simulink model "afe_inv_psm_with_hf_models"  (R2026a)
settings: Solver=ode23tb  StopTime=simlength  FixedStep=tc  MaxStep=glb_time.tc
values from neighbouring files (symbols this model uses):
  afe_ctrl = ctrl_afe_setup(glb_time.ts_afe, grid_emu.omega_grid_nom)    [init_model.m]
  afe_pwm_phase_shift_mod1 = 0    [init_model.m]
  CTRPIFF_CLIP_RELEASE = 0.001    [init_model.m]
  DThs_init = 0    [init_model.m]
  filters = setup_global_filters(glb_time.ts_afe, glb_time.ts_inv, glb_time.ts_dab, glb_time.tc)    [init_model.m]
  frt_data = frt_settings(test_index, test_subindex, asymmetric_error_type,      enable_frt_1, enable_frt_2, start_time_LVRT, deepPOSxi, deepPOSeta, deepNEGxi, deepNEGeta)    [init_model.m]
  glb_time = timing_setup(fpwm_afe, trgo_afe, fpwm_inv, trgo_inv, fpwm_single_phase_inv, trgo_single_phase_inv, fpwm_dab, trgo_dab,      fpwm_psfbc, trgo_psfbc, fpwm_isop_rail, trgo_isop_rail, fpwm_cllc, trgo_cllc, t_measure, tc_factor, tc_decimation, delay_pwm, dead_time_afe,      dead_time_inv, dead_time_single_phase_inv, dead_time_dab, dead_time_psfbc, dead_time_isop_rail, dead_time_cllc)    [init_model.m]
  grid_emu = grid_three_phase_emulator('Dyn11', delta_star, grid_nominal_power, application_voltage, us1, us2, fgrid,                  eq_grid_inductance, eq_grid_resistance, eta, ucc, i1m, p_iron, n1, n2, core_area, core_length, mur,                  up_xi_pu_ref, up_eta_pu_ref, un_xi_pu_ref, un_eta_pu_ref)    [init_model.m]
  i_react_pos_ref_2 = -ixi_ref_mod1*tan(acos(0.95))    [init_model.m]
  i_react_pos_ref_3 = ixi_ref_mod1*tan(acos(0.95))    [init_model.m]
  inv_pwm_phase_shift_mod1 = 0    [init_model.m]
  ixi_ref_mod1 = -0.85    [init_model.m]
  ki_align = 18    [init_model.m]
  kp_align = 0.25    [init_model.m]
  lim_down_align = -0.05    [init_model.m]
  lim_up_align = 0.05    [init_model.m]
  mavarage_filter_frequency_base_order = 2    [init_model.m]
  omega_m_sim = psm.omega_m_bez    [init_model.m]
  psm = psm_calculus_with_variants(application_voltage)    [init_model.m]
  psm_ctrl = ctrl_pmsm_setup(glb_time.ts_inv, psm.omega_bez, u_psm_scale, psm.Jm_norm)    [init_model.m]
  rms_tc = rms_filter_setup(rms_tc_obj)    [init_model.m]
  simlength = 1.75    [init_model.m]
  Tambient = 40    [init_model.m]
  time_aux_power_supply_fault = 1e3    (= 1000)    [init_model.m]
  time_gain_afe_module_1 = 1.0002    [init_model.m]
  time_gain_inv_module_2 = 1.001    [init_model.m]
  time_i_react_pos_ref_1 = start_time_LVRT + error_length + 0.335    [init_model.m]
  time_i_react_pos_ref_2 = time_i_react_pos_ref_1 + 0.5    (= 0.5)    [init_model.m]
  time_start_motor_control = 0.25    [init_model.m]
  torque_overload_factor = 1    [init_model.m]
  u_cm_comp_mod1 = 0    [init_model.m]
  u_psm_scale_ekf = sqrt(3)/2 * 2/3 * hwdata.inv.udc_nom/psm.ubez    [init_model.m]
undefined symbols (not defined in the file or in its folder): hf_power_cable_model, hwdata, magnitude, omega_m_bez, rpm_base, torque_base
libraries: fl_lib x136, nesl_utility x57, moving_average_filter x10, moving_average_filter_cc x8, ee_lib x5, sl_discontinuities x3, single_phase_transformer_lib x3, linear_double_integrator_observer_ccaller x2, discrete_time_low_pass_filter x2, threephase_inductor_lib x2, three_phase_pwm_modulator x2, three_phase_inverter_ideal_switch_based_model x2
(part 2 of 10)

== system afe_inv_psm_with_hf_models/grid/grid_emulator ==
  3ph_Dyg : Subsystem
  Bus Selector : BusSelector  OutputSignals=ua_grid_emu,ub_grid_emu,uc_grid_emu
  Bus Selector1 : BusSelector  OutputSignals=gamma_grid_emulator,omega_grid_emulator
  Controlled Voltage Source : fl_lib/Electrical/Electrical Sources/Controlled Voltage Source
  Controlled Voltage Source1 : fl_lib/Electrical/Electrical Sources/Controlled Voltage Source
  Controlled Voltage Source2 : fl_lib/Electrical/Electrical Sources/Controlled Voltage Source
  Electrical Reference : fl_lib/Electrical/Electrical Elements/Electrical Reference
  Simulink-PS Converter : nesl_utility/Simulink-PS Converter  PhysicalDomain=network_engine_domain  SubClassName=ps_input  LeftPortType=input  RightPortType=output  PseudoPeriodic=off  Frequencies=[]  NoiseDistribution=none  NoiseParameters=[]  Unit=V  AffineConversion=on  FilteringAndDerivatives=provide  SimscapeFilterOrder=1  InputFilterTimeConstant=0.001  UdotUserProvided=0
  Simulink-PS Converter1 : nesl_utility/Simulink-PS Converter  PhysicalDomain=network_engine_domain  SubClassName=ps_input  LeftPortType=input  RightPortType=output  PseudoPeriodic=off  Frequencies=[]  NoiseDistribution=none  NoiseParameters=[]  Unit=V  AffineConversion=on  FilteringAndDerivatives=provide  SimscapeFilterOrder=1  InputFilterTimeConstant=0.001  UdotUserProvided=0
  Simulink-PS Converter2 : nesl_utility/Simulink-PS Converter  PhysicalDomain=network_engine_domain  SubClassName=ps_input  LeftPortType=input  RightPortType=output  PseudoPeriodic=off  Frequencies=[]  NoiseDistribution=none  NoiseParameters=[]  Unit=V  AffineConversion=on  FilteringAndDerivatives=provide  SimscapeFilterOrder=1  InputFilterTimeConstant=0.001  UdotUserProvided=0
  Solver Configuration : nesl_utility/Solver Configuration  PhysicalDomain=network_engine_domain  SubClassName=solver  LeftPortType=input  RightPortType=generic  Tones=[]  Harmonics=[]  SimulateNoise=off  Profile=off  UseLocalSampling=off  EnableSwitchedLinearOptims=on  FrequencyDomain=off  UseCCode=off  RelTol=0.001  AbsTol=0.001  MinStep=1e-09  ToWorkspace=off  RevertToSquareIcSolve=off  NumHomotopyIterations=100  PhasorMode=off  PhasorModeNumHarmonics=1  ConsistencySolver=NEWTON_FTOL  CanonicalOrdering=UNORDERED  OptimizeIntermediates=UNOPTIMIZED  IndexReductionMethod=DerivativeReplacement  DoDC=on  ResidualTolerance=1e-09  ConsistencyTolSource=GLOBAL  ConsistencyAbsTol=0.001  ConsistencyRelTol=0.001  ConsistencyTolFactor=0.001  UseLocalSolver=on  LocalSolverChoice=NE_BACKWARD_EULER_ADVANCER  ResolveIndetEquations=on  FunctionEvalNumThread=1  LocalSolverSampleTime=glb_time.tc  DoFixedCost=on  MaxNonlinIter=nonlinear_iterations  MaxModeIter=2  ComputeImpulses=off  ImpulseIterations=2  LinearAlgebra=auto  LinearAlgebraNumThread=0  EquationFormulation=NE_TIME_EF  DelaysMemoryBudget=1024  AutomaticFiltering=on  FilteringTimeConstant=0.001  PartitionStorageMethod=AS_NEEDED  PartitionMemoryBudget=1024  PartitionMethod=ROBUST  MultibodyUseLocalSolver=off  MultibodyLocalSolverChoice=ODE1  MultibodyLocalSolverSampleTime=0.001
  three_phase_voltage_source_with_frt_emulator : three_phase_voltage_with_frt_emulator/three_phase_voltage_source_with_frt_emulator  nominal_frequency_m=grid_emu.fgrid_nom  nominal_voltage_m=grid_emu.us_primary_nom  Vemu_ref_norm_m=grid_emu.Vemu_ref_norm  vp_xi_pu_m=grid_emu.up_xi_pu_ref  vp_eta_pu_m=grid_emu.up_eta_pu_ref  vn_xi_pu_m=grid_emu.un_xi_pu_ref  vn_eta_pu_m=grid_emu.un_eta_pu_ref  Am=filters.afe.SOF_50Hz.ss_c.A  Bm=filters.afe.SOF_50Hz.ss_c.B  Cm=filters.afe.SOF_50Hz.ss_c.C  enable_frt_1_m=frt_data.enable_frt_1  enable_frt_2_m=frt_data.enable_frt_2  start_time_LVRT_m=frt_data.start_time_LVRT  end_time_LVRT_m=frt_data.end_time_LVRT  deepPOSxi_m=frt_data.deepPOSxi  deepPOSeta_m=frt_data.deepPOSeta  deepNEGxi_m=frt_data.deepNEGxi  deepNEGeta_m=frt_data.deepNEGeta  Amplitude_U_m=frt_data.Amplitude_U  Amplitude_V_m=frt_data.Amplitude_V  Amplitude_W_m=frt_data.Amplitude_W  t_ramp_m=frt_data.t_ramp  Phase_shift_m=frt_data.Phase_shift
  threephase_vi_measures : Subsystem
  u1 : PMIOPort  Side=Right
  u2 : PMIOPort  Port=2  Side=Right
  u3 : PMIOPort  Port=3  Side=Right
  tag scope: gamma_grid_emulator=global, omega_grid_emulator=global
  wires:
  Bus Selector1/2 -> [omega_grid_emulator]  "<omega_grid_emulator>"
  Bus Selector1/1 -> [gamma_grid_emulator]  "<gamma_grid_emulator>"
  Bus Selector/2 -> Simulink-PS Converter1/1  "<ub_grid_emu>"
  Bus Selector/3 -> Simulink-PS Converter2/1  "<uc_grid_emu>"
  three_phase_voltage_source_with_frt_emulator/1 -> Bus Selector1/1, Bus Selector/1
  Bus Selector/1 -> Simulink-PS Converter/1  "<ua_grid_emu>"
  connections:
  Simulink-PS Converter/RConn1 -- Controlled Voltage Source/RConn1
  Simulink-PS Converter1/RConn1 -- Controlled Voltage Source1/RConn1
  Simulink-PS Converter2/RConn1 -- Controlled Voltage Source2/RConn1
  Electrical Reference/LConn1 -- Controlled Voltage Source/RConn2 -- Controlled Voltage Source1/RConn2 -- Controlled Voltage Source2/RConn2 -- Solver Configuration/RConn1
  3ph_Dyg/RConn1 -- u1/RConn1
  3ph_Dyg/RConn2 -- u2/RConn1
  3ph_Dyg/RConn3 -- u3/RConn1
  3ph_Dyg/LConn1 -- threephase_vi_measures/RConn1
  3ph_Dyg/LConn2 -- threephase_vi_measures/RConn2
  3ph_Dyg/LConn3 -- threephase_vi_measures/RConn3
  Controlled Voltage Source/LConn1 -- threephase_vi_measures/LConn1
  Controlled Voltage Source1/LConn1 -- threephase_vi_measures/LConn2
  Controlled Voltage Source2/LConn1 -- threephase_vi_measures/LConn3

== system afe_inv_psm_with_hf_models/grid/threephase_vi_measures ==
  Bus Creator : BusCreator  Inputs=6
  Current Sensor : fl_lib/Electrical/Electrical Sensors/Current Sensor
  Current Sensor1 : fl_lib/Electrical/Electrical Sensors/Current Sensor
  Current Sensor2 : fl_lib/Electrical/Electrical Sensors/Current Sensor
  Electrical Reference1 : fl_lib/Electrical/Electrical Elements/Electrical Reference
  Selector : Selector  InputPortWidth=6  IndexOptions=Index vector (dialog)  Indices=[1 2 3]  OutputSizes=1
  Selector1 : Selector  InputPortWidth=6  IndexOptions=Index vector (dialog)  Indices=[4 5 6]  OutputSizes=1
  Voltage Sensor : fl_lib/Electrical/Electrical Sensors/Voltage Sensor
  Voltage Sensor1 : fl_lib/Electrical/Electrical Sensors/Voltage Sensor
  Voltage Sensor2 : fl_lib/Electrical/Electrical Sensors/Voltage Sensor
  ia_grid : nesl_utility/PS-Simulink Converter  PhysicalDomain=network_engine_domain  SubClassName=ps_output  LeftPortType=input  RightPortType=output  PseudoPeriodic=off  Frequencies=[]  VectorFormat=1-D array  Unit=A  AffineConversion=off
  ib_grid : nesl_utility/PS-Simulink Converter  PhysicalDomain=network_engine_domain  SubClassName=ps_output  LeftPortType=input  RightPortType=output  PseudoPeriodic=off  Frequencies=[]  VectorFormat=1-D array  Unit=A  AffineConversion=off
  ic_grid : nesl_utility/PS-Simulink Converter  PhysicalDomain=network_engine_domain  SubClassName=ps_output  LeftPortType=input  RightPortType=output  PseudoPeriodic=off  Frequencies=[]  VectorFormat=1-D array  Unit=A  AffineConversion=off
  ig_abc/ug_abc : Scope  NumInputPorts=2
      settings: SampleTime=glb_time.tc  ActiveDisplayYMinimum=-728.92703752654245  ActiveDisplayYMaximum=734.90808013997  DataLoggingVariableName=ScopeData2
  ua_grid : nesl_utility/PS-Simulink Converter  PhysicalDomain=network_engine_domain  SubClassName=ps_output  LeftPortType=input  RightPortType=output  PseudoPeriodic=off  Frequencies=[]  VectorFormat=1-D array  Unit=V  AffineConversion=off
  ub_grid : nesl_utility/PS-Simulink Converter  PhysicalDomain=network_engine_domain  SubClassName=ps_output  LeftPortType=input  RightPortType=output  PseudoPeriodic=off  Frequencies=[]  VectorFormat=1-D array  Unit=V  AffineConversion=off
  uc_grid : nesl_utility/PS-Simulink Converter  PhysicalDomain=network_engine_domain  SubClassName=ps_output  LeftPortType=input  RightPortType=output  PseudoPeriodic=off  Frequencies=[]  VectorFormat=1-D array  Unit=V  AffineConversion=off
  Ua : PMIOPort  Side=Left
  ua : PMIOPort  Port=2  Side=Right
  Ub : PMIOPort  Port=3  Side=Left
  ub : PMIOPort  Port=4  Side=Right
  Uc : PMIOPort  Port=5  Side=Left
  uc : PMIOPort  Port=6  Side=Right
  tag scope: ig_abc=global, ug_abc=global
  wires:
  Bus Creator/1 -> Selector1/1, Selector/1  "vi_data"
  Selector/1 -> [ug_abc]
  ib_grid/1 -> Bus Creator/5  "ib"
  ia_grid/1 -> Bus Creator/4  "ia"
  ic_grid/1 -> Bus Creator/6  "ic"
  ua_grid/1 -> Bus Creator/1  "ua"
  ub_grid/1 -> Bus Creator/2  "ub"
  uc_grid/1 -> Bus Creator/3  "uc"
  Selector1/1 -> [ig_abc]
  [ug_abc] -> ig_abc/ug_abc/2  "ug_abc(line)"
  [ig_abc] -> ig_abc/ug_abc/1  "ig_abc(line)"
  connections:
  Current Sensor1/LConn1 -- Ub/RConn1 -- Voltage Sensor1/LConn1
  Electrical Reference1/LConn1 -- Voltage Sensor/RConn2 -- Voltage Sensor2/RConn2 -- Voltage Sensor1/RConn2
  Voltage Sensor/RConn1 -- ua_grid/LConn1
  Current Sensor/RConn2 -- ua/RConn1
  Voltage Sensor1/RConn1 -- ub_grid/LConn1
  Voltage Sensor2/LConn1 -- Current Sensor2/LConn1 -- Uc/RConn1
  Current Sensor/LConn1 -- Ua/RConn1 -- Voltage Sensor/LConn1
  Current Sensor1/RConn2 -- ub/RConn1
  Voltage Sensor2/RConn1 -- uc_grid/LConn1
  ib_grid/LConn1 -- Current Sensor1/RConn1
  ia_grid/LConn1 -- Current Sensor/RConn1
  ic_grid/LConn1 -- Current Sensor2/RConn1
  Current Sensor2/RConn2 -- uc/RConn1

== system afe_inv_psm_with_hf_models/inverter_measurement_sim/high_frequency_power_cable ==
  To Workspace21 : ToWorkspace  VariableName=is_uvw_cm_sim  SampleTime=glb_time.tc
      settings: MaxDataPoints=glb_time.Nc
  To Workspace22 : ToWorkspace  VariableName=udc_pgnd_sim  SampleTime=glb_time.tc
      settings: MaxDataPoints=glb_time.Nc
  To Workspace23 : ToWorkspace  VariableName=udc_ngnd_sim  SampleTime=glb_time.tc
      settings: MaxDataPoints=glb_time.Nc
  To Workspace24 : ToWorkspace  VariableName=iz_power_cable_drive_side_sim  SampleTime=glb_time.tc
      settings: MaxDataPoints=glb_time.Nc
  To Workspace25 : ToWorkspace  VariableName=i_power_cable_drive_side_sim  SampleTime=glb_time.tc
      settings: MaxDataPoints=glb_time.Nc
  To Workspace26 : ToWorkspace  VariableName=u_power_cable_drive_side_sim  SampleTime=glb_time.tc
      settings: MaxDataPoints=glb_time.Nc
  To Workspace27 : ToWorkspace  VariableName=iz_power_cable_machine_side_sim  SampleTime=glb_time.tc
      settings: MaxDataPoints=glb_time.Nc
  To Workspace28 : ToWorkspace  VariableName=i_power_cable_machine_side_sim  SampleTime=glb_time.tc
      settings: MaxDataPoints=glb_time.Nc
  To Workspace29 : ToWorkspace  VariableName=u_power_cable_machine_side_sim  SampleTime=glb_time.tc
      settings: MaxDataPoints=glb_time.Nc
  wires:
  [i_power_cable_drive_side] -> To Workspace25/1  "i_power_cable_drive_side"
  [is_uvw_cm] -> To Workspace21/1  "is_uvw_cm"
  [iz_power_cable_machine_side] -> To Workspace27/1  "iz_power_cable_machine_side"
  [iz_power_cable_drive_side] -> To Workspace24/1  "iz_power_cable_drive_side"
  [i_power_cable_machine_side] -> To Workspace28/1  "i_power_cable_machine_side"
  [udc_pgnd] -> To Workspace22/1  "udc_pgnd"
  [u_power_cable_drive_side] -> To Workspace26/1  "u_power_cable_drive_side"
  [udc_ngnd] -> To Workspace23/1  "udc_ngnd"
  [u_power_cable_machine_side] -> To Workspace29/1  "u_power_cable_machine_side"

== system afe_inv_psm_with_hf_models/inverter_measurement_sim/module_1 ==
  To Workspace12 : ToWorkspace  VariableName=ileg_dc_inv_sim_mod1  SampleTime=glb_time.tc
      settings: MaxDataPoints=glb_time.Nc
  To Workspace14 : ToWorkspace  VariableName=is_uvw_sim_mod1  SampleTime=glb_time.tc
      settings: MaxDataPoints=glb_time.Nc
  To Workspace15 : ToWorkspace  VariableName=us_uvw_sim_mod1  SampleTime=glb_time.tc
      settings: MaxDataPoints=glb_time.Nc
  wires:
  [us_uvw_pu] -> To Workspace15/1
  [ileg_dc_inv_mod1] -> To Workspace12/1
  [is_uvw_pu] -> To Workspace14/1

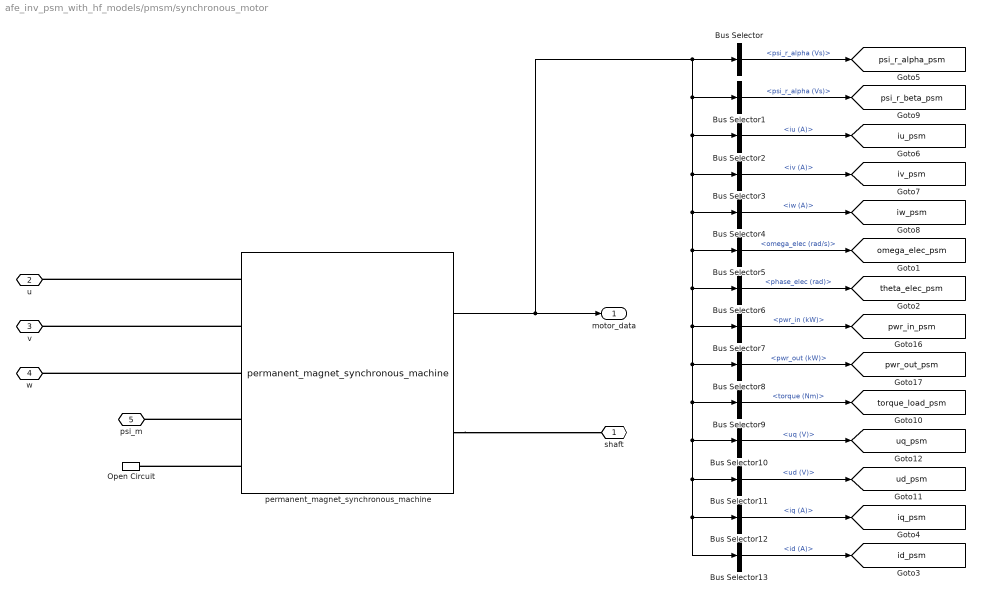
== system afe_inv_psm_with_hf_models/pmsm/synchronous_motor ==
  Bus Selector : BusSelector  OutputSignals=psi_r_alpha (Vs)
  Bus Selector1 : BusSelector  OutputSignals=psi_r_alpha (Vs)
  Bus Selector10 : BusSelector  OutputSignals=uq (V)
  Bus Selector11 : BusSelector  OutputSignals=ud (V)
  Bus Selector12 : BusSelector  OutputSignals=iq (A)
  Bus Selector13 : BusSelector  OutputSignals=id (A)
  Bus Selector2 : BusSelector  OutputSignals=iu (A)
  Bus Selector3 : BusSelector  OutputSignals=iv (A)
  Bus Selector4 : BusSelector  OutputSignals=iw (A)
  Bus Selector5 : BusSelector  OutputSignals=omega_elec (rad/s)
  Bus Selector6 : BusSelector  OutputSignals=phase_elec (rad)
  Bus Selector7 : BusSelector  OutputSignals=pwr_in (kW)
  Bus Selector8 : BusSelector  OutputSignals=pwr_out (kW)
  Bus Selector9 : BusSelector  OutputSignals=torque (Nm)
  Open Circuit : fl_lib/Electrical/Electrical Elements/Open Circuit  v_specify=off  v_priority=None  v=0 V  v_nominal_specify=off  v_nominal_value=1  v_nominal_unit=V
  permanent_magnet_synchronous_machine : permanent_magnet_synchronous_machine/permanent_magnet_synchronous_machine  pp=psm.number_poles  psi_m=psm.psi_m  Lmu=psm.Lmu  La=psm.La_m  Lb=psm.Lb_m  Rs=psm.Rs_m  Jm=psm.Jm_m  b_linear=psm.load_friction_m  b_quadratic=0  h5_percent=0  h7_percent=0  psi_r_u_init=psm.psi_m  psi_r_v_init=-psm.psi_m/2  psi_r_w_init=-psm.psi_m/2  omega_init=0  phase_init=0  angle_error=0
  shaft : PMIOPort  Side=Right
  u : PMIOPort  Port=2  Side=Left
  v : PMIOPort  Port=3  Side=Left
  w : PMIOPort  Port=4  Side=Left
  psi_m : PMIOPort  Port=5  Side=Left
  motor_data : Outport
  tag scope: id_psm=global, iq_psm=global, iu_psm=global, iv_psm=global, iw_psm=global, omega_elec_psm=global, psi_r_alpha_psm=global, psi_r_beta_psm=global, pwr_in_psm=global, pwr_out_psm=global, theta_elec_psm=global, torque_load_psm=global, ud_psm=global, uq_psm=global
  wires:
  permanent_magnet_synchronous_machine/1 -> Bus Selector8/1, Bus Selector10/1, Bus Selector11/1, Bus Selector12/1, Bus Selector13/1, Bus Selector9/1, Bus Selector7/1, Bus Selector6/1, Bus Selector5/1, Bus Selector4/1, Bus Selector3/1, Bus Selector2/1, Bus Selector1/1, Bus Selector/1, motor_data/1
  Bus Selector/1 -> [psi_r_alpha_psm]  "<psi_r_alpha (Vs)>"
  Bus Selector1/1 -> [psi_r_beta_psm]  "<psi_r_alpha (Vs)>"
  Bus Selector2/1 -> [iu_psm]  "<iu (A)>"
  Bus Selector3/1 -> [iv_psm]  "<iv (A)>"
  Bus Selector4/1 -> [iw_psm]  "<iw (A)>"
  Bus Selector5/1 -> [omega_elec_psm]  "<omega_elec (rad/s)>"
  Bus Selector6/1 -> [theta_elec_psm]  "<phase_elec (rad)>"
  Bus Selector7/1 -> [pwr_in_psm]  "<pwr_in (kW)>"
  Bus Selector8/1 -> [pwr_out_psm]  "<pwr_out (kW)>"
  Bus Selector9/1 -> [torque_load_psm]  "<torque (Nm)>"
  Bus Selector10/1 -> [uq_psm]  "<uq (V)>"
  Bus Selector11/1 -> [ud_psm]  "<ud (V)>"
  Bus Selector12/1 -> [iq_psm]  "<iq (A)>"
  Bus Selector13/1 -> [id_psm]  "<id (A)>"
  connections:
  permanent_magnet_synchronous_machine/RConn1 -- shaft/RConn1
  permanent_magnet_synchronous_machine/LConn1 -- u/RConn1
  permanent_magnet_synchronous_machine/LConn2 -- v/RConn1
  permanent_magnet_synchronous_machine/LConn3 -- w/RConn1
  permanent_magnet_synchronous_machine/LConn4 -- psi_m/RConn1
  permanent_magnet_synchronous_machine/LConn5 -- Open Circuit/LConn1

== system afe_inv_psm_with_hf_models/power_cables_and_psm_high_frequency_models/Subsystem ==
  Electrical Reference : fl_lib/Electrical/Electrical Elements/Electrical Reference
  Electrical Reference1 : fl_lib/Electrical/Electrical Elements/Electrical Reference
  Transmission Line : ee_lib/Passive/Lines/Transmission Line  model_type=ee.enum.lines.modelType.LumpedParameterPiSection  LC_param=ee.enum.lines.parameterization.IndAndCap  TD=5 ns  Z0_delay_based=50 Ohm  Z0=50 Ohm  freq=50 Hz  Ll=220 uH/m  L=220 uH/m  C=0.3 uF/m  R=0.25 Ohm/m  G=5e-6 S/m  LEN=120 m  N=1
  Transmission Line1 : ee_lib/Passive/Lines/Transmission Line  model_type=ee.enum.lines.modelType.LumpedParameterPiSection  LC_param=ee.enum.lines.parameterization.IndAndCap  TD=5 ns  Z0_delay_based=50 Ohm  Z0=50 Ohm  freq=50 Hz  Ll=220 uH/m  L=220 uH/m  C=0.3 uF/m  R=0.25 Ohm/m  G=5e-6 S/m  LEN=120 m  N=1
  Transmission Line2 : ee_lib/Passive/Lines/Transmission Line  model_type=ee.enum.lines.modelType.LumpedParameterPiSection  LC_param=ee.enum.lines.parameterization.IndAndCap  TD=5 ns  Z0_delay_based=50 Ohm  Z0=50 Ohm  freq=50 Hz  Ll=220 uH/m  L=220 uH/m  C=0.3 uF/m  R=0.25 Ohm/m  G=5e-6 S/m  LEN=120 m  N=1
  Conn1 : PMIOPort  Side=Left
  Conn2 : PMIOPort  Port=2  Side=Right
  Conn3 : PMIOPort  Port=3  Side=Left
  Conn4 : PMIOPort  Port=4  Side=Right
  Conn5 : PMIOPort  Port=5  Side=Left
  Conn6 : PMIOPort  Port=6  Side=Right
  connections:
  Transmission Line/LConn1 -- Conn1/RConn1
  Electrical Reference/LConn1 -- Transmission Line/LConn2 -- Transmission Line1/LConn2 -- Transmission Line2/LConn2
  Conn6/RConn1 -- Transmission Line2/RConn1
  Transmission Line1/LConn1 -- Conn3/RConn1
  Transmission Line/RConn2 -- Transmission Line1/RConn2 -- Transmission Line2/RConn2 -- Electrical Reference1/LConn1
  Transmission Line2/LConn1 -- Conn5/RConn1
  Conn4/RConn1 -- Transmission Line1/RConn1
  Conn2/RConn1 -- Transmission Line/RConn1

== system afe_inv_psm_with_hf_models/power_cables_and_psm_high_frequency_models/Subsystem1 ==
  Electrical Reference : fl_lib/Electrical/Electrical Elements/Electrical Reference
  Electrical Reference1 : fl_lib/Electrical/Electrical Elements/Electrical Reference
  Transmission Line (Three-Phase) : ee_lib/Passive/Lines/Transmission Line (Three-Phase)  port_option=ee.enum.threePhasePort.expanded  length=0.12 km  freq=60 Hz  prm=ee.enum.lines.parameterization3ph.physicalLineParam  R=0.25 Ohm/km  Rm=0 Ohm/km  L=0.25 mH/km  M=0.22 mH/km  Cl=0.1 uF/km  Cg=0.3 uF/km  Rpos=0.01 Ohm/km  Rzero=0.04 Ohm/km  Lpos=0.4 mH/km  Lzero=0.7 mH/km  Cpos=1 uF/km  Czero=0.1 uF/km  ModelTwoSections=ee.enum.enable.no  N=1  InterfacePosition=0.5 km  N1sec=1  N2sec=1  Access_ground=ee.enum.enable.no  R_parasitic=1e-6 Ohm  G_parasitic=1e-6 1/Ohm
  Conn1 : PMIOPort  Side=Left
  Conn2 : PMIOPort  Port=2  Side=Right
  Conn3 : PMIOPort  Port=3  Side=Left
  Conn4 : PMIOPort  Port=4  Side=Right
  Conn5 : PMIOPort  Port=5  Side=Left
  Conn6 : PMIOPort  Port=6  Side=Right
  connections:
  Transmission Line (Three-Phase)/LConn4 -- Electrical Reference/LConn1
  Transmission Line (Three-Phase)/RConn1 -- Conn2/RConn1
  Transmission Line (Three-Phase)/RConn3 -- Conn6/RConn1
  Transmission Line (Three-Phase)/RConn2 -- Conn4/RConn1
  Transmission Line (Three-Phase)/LConn3 -- Conn5/RConn1
  Transmission Line (Three-Phase)/RConn4 -- Electrical Reference1/LConn1
  Transmission Line (Three-Phase)/LConn1 -- Conn1/RConn1
  Transmission Line (Three-Phase)/LConn2 -- Conn3/RConn1

== system afe_inv_psm_with_hf_models/power_cables_and_psm_high_frequency_models/power_cable_model_1 ==
  parasitic_lump_1 : Subsystem
  parasitic_lump_2 : Subsystem
  u1 : PMIOPort  Side=Left
  u2 : PMIOPort  Port=2  Side=Right
  connections:
  parasitic_lump_1/LConn1 -- u1/RConn1
  parasitic_lump_2/RConn1 -- u2/RConn1
  parasitic_lump_1/RConn1 -- parasitic_lump_2/LConn1

== system afe_inv_psm_with_hf_models/power_cables_and_psm_high_frequency_models/power_cable_model_2 ==
  parasitic_lump_1 : Subsystem
  parasitic_lump_2 : Subsystem
  u1 : PMIOPort  Side=Left
  u2 : PMIOPort  Port=2  Side=Right
  connections:
  parasitic_lump_1/RConn1 -- parasitic_lump_2/LConn1
  parasitic_lump_2/RConn1 -- u2/RConn1
  parasitic_lump_1/LConn1 -- u1/RConn1

== system afe_inv_psm_with_hf_models/power_cables_and_psm_high_frequency_models/power_cable_model_3 ==
  parasitic_lump_1 : Subsystem
  parasitic_lump_2 : Subsystem
  u1 : PMIOPort  Side=Left
  u2 : PMIOPort  Port=2  Side=Right
  connections:
  parasitic_lump_1/LConn1 -- u1/RConn1
  parasitic_lump_2/RConn1 -- u2/RConn1
  parasitic_lump_1/RConn1 -- parasitic_lump_2/LConn1

== system afe_inv_psm_with_hf_models/power_cables_and_psm_high_frequency_models/threephase_vi_measures_driver_side ==
  Bus Creator : BusCreator  Inputs=6
  Current Sensor : fl_lib/Electrical/Electrical Sensors/Current Sensor
  Current Sensor1 : fl_lib/Electrical/Electrical Sensors/Current Sensor
  Current Sensor2 : fl_lib/Electrical/Electrical Sensors/Current Sensor
  Electrical Reference1 : fl_lib/Electrical/Electrical Elements/Electrical Reference
  Selector : Selector  InputPortWidth=6  IndexOptions=Index vector (dialog)  Indices=[1 2 3]  OutputSizes=1
  Selector1 : Selector  InputPortWidth=6  IndexOptions=Index vector (dialog)  Indices=[4 5 6]  OutputSizes=1
  Sum : Sum  Inputs=+++
  Voltage Sensor : fl_lib/Electrical/Electrical Sensors/Voltage Sensor
  Voltage Sensor1 : fl_lib/Electrical/Electrical Sensors/Voltage Sensor
  Voltage Sensor2 : fl_lib/Electrical/Electrical Sensors/Voltage Sensor
  iu_inv : nesl_utility/PS-Simulink Converter  PhysicalDomain=network_engine_domain  SubClassName=ps_output  LeftPortType=input  RightPortType=output  PseudoPeriodic=off  Frequencies=[]  VectorFormat=1-D array  Unit=A  AffineConversion=off
  iv_inv : nesl_utility/PS-Simulink Converter  PhysicalDomain=network_engine_domain  SubClassName=ps_output  LeftPortType=input  RightPortType=output  PseudoPeriodic=off  Frequencies=[]  VectorFormat=1-D array  Unit=A  AffineConversion=off
  iw_inv : nesl_utility/PS-Simulink Converter  PhysicalDomain=network_engine_domain  SubClassName=ps_output  LeftPortType=input  RightPortType=output  PseudoPeriodic=off  Frequencies=[]  VectorFormat=1-D array  Unit=A  AffineConversion=off
  uu_inv : nesl_utility/PS-Simulink Converter  PhysicalDomain=network_engine_domain  SubClassName=ps_output  LeftPortType=input  RightPortType=output  PseudoPeriodic=off  Frequencies=[]  VectorFormat=1-D array  Unit=V  AffineConversion=off
  uv_inv : nesl_utility/PS-Simulink Converter  PhysicalDomain=network_engine_domain  SubClassName=ps_output  LeftPortType=input  RightPortType=output  PseudoPeriodic=off  Frequencies=[]  VectorFormat=1-D array  Unit=V  AffineConversion=off
  uw_inv : nesl_utility/PS-Simulink Converter  PhysicalDomain=network_engine_domain  SubClassName=ps_output  LeftPortType=input  RightPortType=output  PseudoPeriodic=off  Frequencies=[]  VectorFormat=1-D array  Unit=V  AffineConversion=off
  Uu : PMIOPort  Side=Left
  uu : PMIOPort  Port=2  Side=Right
  Uv : PMIOPort  Port=3  Side=Left
  uv : PMIOPort  Port=4  Side=Right
  Uw : PMIOPort  Port=5  Side=Left
  uw : PMIOPort  Port=6  Side=Right
  tag scope: i_power_cable_drive_side=global, iz_power_cable_drive_side=global, u_power_cable_drive_side=global
  wires:
  Bus Creator/1 -> Selector/1, Selector1/1  "vi_data"
  Selector/1 -> [u_power_cable_drive_side]
  iv_inv/1 -> Bus Creator/5, Sum/2  "iv_inv"
  iu_inv/1 -> Bus Creator/4, Sum/1  "iu_inv"
  iw_inv/1 -> Bus Creator/6, Sum/3  "iw_inv"
  uu_inv/1 -> Bus Creator/1  "uu_inv"
  uv_inv/1 -> Bus Creator/2  "uv_inv"
  uw_inv/1 -> Bus Creator/3  "uw_inv"
  Selector1/1 -> [i_power_cable_drive_side]
  Sum/1 -> [iz_power_cable_drive_side]
  connections:
  Current Sensor1/LConn1 -- Uv/RConn1 -- Voltage Sensor1/LConn1
  Electrical Reference1/LConn1 -- Voltage Sensor/RConn2 -- Voltage Sensor2/RConn2 -- Voltage Sensor1/RConn2
  Voltage Sensor/RConn1 -- uu_inv/LConn1
  Current Sensor/RConn2 -- uu/RConn1
  Voltage Sensor1/RConn1 -- uv_inv/LConn1
  Voltage Sensor2/LConn1 -- Uw/RConn1 -- Current Sensor2/LConn1
  Current Sensor/LConn1 -- Uu/RConn1 -- Voltage Sensor/LConn1
  Current Sensor1/RConn2 -- uv/RConn1
  Voltage Sensor2/RConn1 -- uw_inv/LConn1
  iv_inv/LConn1 -- Current Sensor1/RConn1
  iu_inv/LConn1 -- Current Sensor/RConn1
  iw_inv/LConn1 -- Current Sensor2/RConn1
  Current Sensor2/RConn2 -- uw/RConn1

== system afe_inv_psm_with_hf_models/power_cables_and_psm_high_frequency_models/threephase_vi_measures_machine_side ==
  Bus Creator : BusCreator  Inputs=6
  Current Sensor : fl_lib/Electrical/Electrical Sensors/Current Sensor
  Current Sensor1 : fl_lib/Electrical/Electrical Sensors/Current Sensor
  Current Sensor2 : fl_lib/Electrical/Electrical Sensors/Current Sensor
  Electrical Reference1 : fl_lib/Electrical/Electrical Elements/Electrical Reference
  Selector : Selector  InputPortWidth=6  IndexOptions=Index vector (dialog)  Indices=[1 2 3]  OutputSizes=1
  Selector1 : Selector  InputPortWidth=6  IndexOptions=Index vector (dialog)  Indices=[4 5 6]  OutputSizes=1
  Sum : Sum  Inputs=+++
  Voltage Sensor : fl_lib/Electrical/Electrical Sensors/Voltage Sensor
  Voltage Sensor1 : fl_lib/Electrical/Electrical Sensors/Voltage Sensor
  Voltage Sensor2 : fl_lib/Electrical/Electrical Sensors/Voltage Sensor
  iu_inv : nesl_utility/PS-Simulink Converter  PhysicalDomain=network_engine_domain  SubClassName=ps_output  LeftPortType=input  RightPortType=output  PseudoPeriodic=off  Frequencies=[]  VectorFormat=1-D array  Unit=A  AffineConversion=off
  iv_inv : nesl_utility/PS-Simulink Converter  PhysicalDomain=network_engine_domain  SubClassName=ps_output  LeftPortType=input  RightPortType=output  PseudoPeriodic=off  Frequencies=[]  VectorFormat=1-D array  Unit=A  AffineConversion=off
  iw_inv : nesl_utility/PS-Simulink Converter  PhysicalDomain=network_engine_domain  SubClassName=ps_output  LeftPortType=input  RightPortType=output  PseudoPeriodic=off  Frequencies=[]  VectorFormat=1-D array  Unit=A  AffineConversion=off
  uu_inv : nesl_utility/PS-Simulink Converter  PhysicalDomain=network_engine_domain  SubClassName=ps_output  LeftPortType=input  RightPortType=output  PseudoPeriodic=off  Frequencies=[]  VectorFormat=1-D array  Unit=V  AffineConversion=off
  uv_inv : nesl_utility/PS-Simulink Converter  PhysicalDomain=network_engine_domain  SubClassName=ps_output  LeftPortType=input  RightPortType=output  PseudoPeriodic=off  Frequencies=[]  VectorFormat=1-D array  Unit=V  AffineConversion=off
  uw_inv : nesl_utility/PS-Simulink Converter  PhysicalDomain=network_engine_domain  SubClassName=ps_output  LeftPortType=input  RightPortType=output  PseudoPeriodic=off  Frequencies=[]  VectorFormat=1-D array  Unit=V  AffineConversion=off
  Uu : PMIOPort  Side=Left
  uu : PMIOPort  Port=2  Side=Right
  Uv : PMIOPort  Port=3  Side=Left
  uv : PMIOPort  Port=4  Side=Right
  Uw : PMIOPort  Port=5  Side=Left
  uw : PMIOPort  Port=6  Side=Right
  tag scope: i_power_cable_machine_side=global, iz_power_cable_machine_side=global, u_power_cable_machine_side=global
  wires:
  Sum/1 -> [iz_power_cable_machine_side]
  Selector1/1 -> [i_power_cable_machine_side]
  uw_inv/1 -> Bus Creator/3  "uw_inv"
  uv_inv/1 -> Bus Creator/2  "uv_inv"
  uu_inv/1 -> Bus Creator/1  "uu_inv"
  iw_inv/1 -> Sum/3, Bus Creator/6  "iw_inv"
  iu_inv/1 -> Sum/1, Bus Creator/4  "iu_inv"
  iv_inv/1 -> Sum/2, Bus Creator/5  "iv_inv"
  Selector/1 -> [u_power_cable_machine_side]
  Bus Creator/1 -> Selector1/1, Selector/1  "vi_data"
  connections:
  Current Sensor2/RConn2 -- uw/RConn1
  iw_inv/LConn1 -- Current Sensor2/RConn1
  iu_inv/LConn1 -- Current Sensor/RConn1
  iv_inv/LConn1 -- Current Sensor1/RConn1
  Voltage Sensor2/RConn1 -- uw_inv/LConn1
  Current Sensor1/RConn2 -- uv/RConn1
  Voltage Sensor/LConn1 -- Uu/RConn1 -- Current Sensor/LConn1
  Current Sensor2/LConn1 -- Uw/RConn1 -- Voltage Sensor2/LConn1
  Voltage Sensor1/RConn1 -- uv_inv/LConn1
  Current Sensor/RConn2 -- uu/RConn1
  Voltage Sensor/RConn1 -- uu_inv/LConn1
  Voltage Sensor1/RConn2 -- Voltage Sensor2/RConn2 -- Voltage Sensor/RConn2 -- Electrical Reference1/LConn1
  Voltage Sensor1/LConn1 -- Uv/RConn1 -- Current Sensor1/LConn1

== system afe_inv_psm_with_hf_models/scopes/cable_effects ==
  Sum : Sum  Inputs=|+-
  cable_effects1 : Scope  NumInputPorts=4
      settings: SampleTime=glb_time.tc  ActiveDisplayYMinimum=-254.85002654941417  ActiveDisplayYMaximum=208.81944946289155  DataLoggingVariableName=ScopeData36
  cable_effects2 : Scope  NumInputPorts=3
      settings: SampleTime=glb_time.tc  ActiveDisplayYMinimum=-1  ActiveDisplayYMaximum=1  DataLoggingVariableName=ScopeData37
  cable_effects3 : Scope  NumInputPorts=4
      settings: SampleTime=glb_time.tc  ActiveDisplayYMinimum=-222.1102318469415  ActiveDisplayYMaximum=212.84276977838644  DataLoggingVariableName=ScopeData35
  rms : Subsystem
  wires:
  [udc_pgnd] -> Sum/1, cable_effects3/2  "udc_pgnd"
  [udc_ngnd] -> Sum/2, cable_effects3/3  "udc_ngnd"
  [is_uvw_cm] -> cable_effects3/1  "is_uvw_cm"
  [i_power_cable_drive_side] -> cable_effects1/2  "i_power_cable_drive_side"
  [u_power_cable_drive_side] -> cable_effects1/3  "u_power_cable_drive_side"
  [iz_power_cable_machine_side] -> cable_effects2/1  "iz_power_cable_machine_side"
  [i_power_cable_machine_side] -> cable_effects2/2  "i_power_cable_machine_side"
  [u_power_cable_machine_side] -> cable_effects2/3  "u_power_cable_machine_side"
  [iz_power_cable_drive_side] -> rms/1(in), cable_effects1/1  "iz_power_cable_drive_side"
  rms/1(out) -> cable_effects1/4  "iz_rms"
  Sum/1 -> cable_effects3/4  "udc"

== system afe_inv_psm_with_hf_models/scopes/grid_afe_side ==
  Gain7 : Gain  Gain=hwdata.afe.ibez
  Gain8 : Gain  Gain=hwdata.afe.ubez
  Gain9 : Gain  Gain=hwdata.afe.ibez
  IEC_power_meter : Scope  NumInputPorts=4
      settings: ActiveDisplayYMinimum=-139946.10544863567  ActiveDisplayYMaximum=229911.63765155774  DataLoggingVariableName=ScopeData14
  i_line_abc/u_line_abc : Scope  NumInputPorts=2
      settings: SampleTime=glb_time.tc  ActiveDisplayYMinimum=-1352.5734119476883  ActiveDisplayYMaximum=1505.395019752161  DataLoggingVariableName=ScopeData20
  idc/udc : Scope  NumInputPorts=2
      settings: SampleTime=glb_time.tc  ActiveDisplayYMinimum=-237.45231016815259  ActiveDisplayYMaximum=320.54398715417091  DataLoggingVariableName=ScopeData23
  ig_abc/ug_abc _mod1 : Scope  NumInputPorts=2
      settings: SampleTime=glb_time.tc  ActiveDisplayYMinimum=-4.4957016262667837  ActiveDisplayYMaximum=4.3239423057982735  DataLoggingVariableName=ScopeData22
  is_abc/us_abc _mod1 : Scope  NumInputPorts=3
      settings: SampleTime=glb_time.tc  ActiveDisplayYMinimum=-2620.8441075302808  ActiveDisplayYMaximum=2310.3545900694107  DataLoggingVariableName=ScopeData21
  udc voltages : Scope  NumInputPorts=2
      settings: SampleTime=glb_time.tc  ActiveDisplayYMinimum=-0.1691941690232826  ActiveDisplayYMaximum=1.5064339432334795  DataLoggingVariableName=ScopeData24
  wires:
  [udc_mod1] -> idc/udc/2  "udc_dclink_mod1"
  [ug_abc_pu_mod1] -> ig_abc/ug_abc _mod1/2  "ug_abc_mod1"
  Gain8/1 -> is_abc/us_abc _mod1/2  "vs_abc_mod1"
  [ic_dclink_mod1] -> idc/udc/1  "ic_dclink_mod1"
  [is_abc_pu_mod1] -> Gain7/1
  [Q1p_global] -> IEC_power_meter/2  "Q1p_global"
  [all_voltages_about_dclink] -> udc voltages/2  "all_voltages_about_dclink"
  Gain7/1 -> is_abc/us_abc _mod1/1  "is_abc_mod1"
  [iz_afe_pu_mod1] -> Gain9/1
  [i_abc_line] -> i_line_abc/u_line_abc/1  "i_abc_line"
  [u_abc_line] -> i_line_abc/u_line_abc/2  "u_abc_line"
  [P1n_global] -> IEC_power_meter/4  "P1n_global"
  [ig_abc_pu_mod1] -> ig_abc/ug_abc _mod1/1  "ig_abc_mod1"
  [vs_abc_pu_mod1] -> Gain8/1
  [vdc_pu_afe_mod1] -> udc voltages/1  "udc"
  Gain9/1 -> is_abc/us_abc _mod1/3  "iz_afe_mod1"
  [Q1n_global] -> IEC_power_meter/1  "Q1n_global"
  [P1p_global] -> IEC_power_meter/3  "P1p_global"

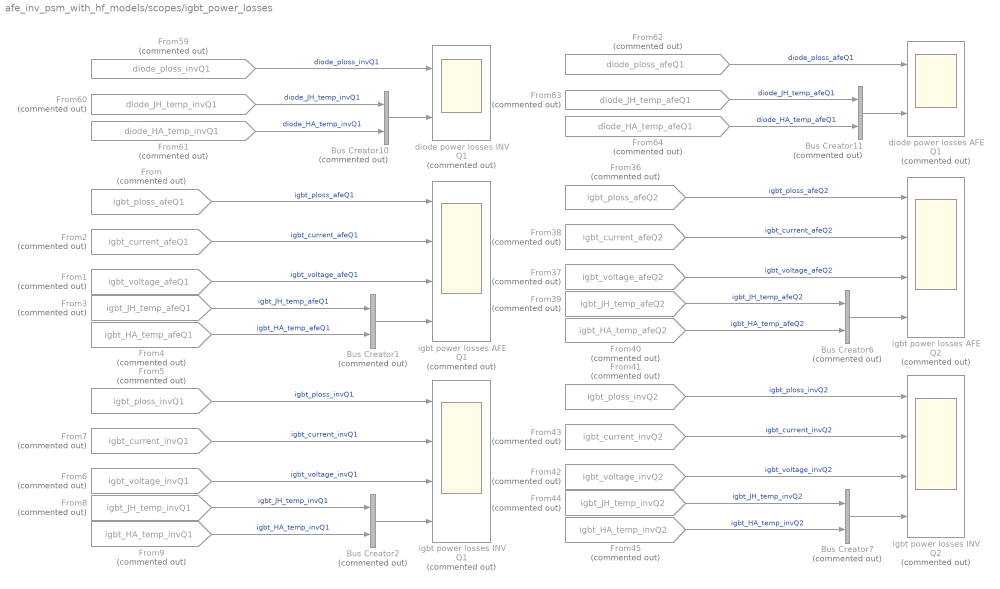
== system afe_inv_psm_with_hf_models/scopes/igbt_power_losses ==
  Bus Creator{1..2,6..7,10..11} (6 alike) : BusCreator  Commented=on  Inputs=2
  From : From  Commented=on  GotoTag=igbt_ploss_afeQ1
  From1 : From  Commented=on  GotoTag=igbt_voltage_afeQ1
  From2 : From  Commented=on  GotoTag=igbt_current_afeQ1
  From3 : From  Commented=on  GotoTag=igbt_JH_temp_afeQ1
  From36 : From  Commented=on  GotoTag=igbt_ploss_afeQ2
  From37 : From  Commented=on  GotoTag=igbt_voltage_afeQ2
  From38 : From  Commented=on  GotoTag=igbt_current_afeQ2
  From39 : From  Commented=on  GotoTag=igbt_JH_temp_afeQ2
  From4 : From  Commented=on  GotoTag=igbt_HA_temp_afeQ1
  From40 : From  Commented=on  GotoTag=igbt_HA_temp_afeQ2
  From41 : From  Commented=on  GotoTag=igbt_ploss_invQ2
  From42 : From  Commented=on  GotoTag=igbt_voltage_invQ2
  From43 : From  Commented=on  GotoTag=igbt_current_invQ2
  From44 : From  Commented=on  GotoTag=igbt_JH_temp_invQ2
  From45 : From  Commented=on  GotoTag=igbt_HA_temp_invQ2
  From5 : From  Commented=on  GotoTag=igbt_ploss_invQ1
  From59 : From  Commented=on  GotoTag=diode_ploss_invQ1
  From6 : From  Commented=on  GotoTag=igbt_voltage_invQ1
  From60 : From  Commented=on  GotoTag=diode_JH_temp_invQ1
  From61 : From  Commented=on  GotoTag=diode_HA_temp_invQ1
  From62 : From  Commented=on  GotoTag=diode_ploss_afeQ1
  From63 : From  Commented=on  GotoTag=diode_JH_temp_afeQ1
  From64 : From  Commented=on  GotoTag=diode_HA_temp_afeQ1
  From7 : From  Commented=on  GotoTag=igbt_current_invQ1
  From8 : From  Commented=on  GotoTag=igbt_JH_temp_invQ1
  From9 : From  Commented=on  GotoTag=igbt_HA_temp_invQ1
  diode power losses AFE Q1 : Scope  Commented=on  NumInputPorts=2
      settings: SampleTime=glb_time.tc  ActiveDisplayYMinimum=-0.87039317174009745  ActiveDisplayYMaximum=7.8312553964690395  DataLoggingVariableName=ScopeData32
  diode power losses INV Q1 : Scope  Commented=on  NumInputPorts=2
      settings: SampleTime=glb_time.tc  ActiveDisplayYMinimum=-1  ActiveDisplayYMaximum=1  DataLoggingVariableName=ScopeData31
  igbt power losses AFE Q1 : Scope  Commented=on  NumInputPorts=4
      settings: SampleTime=glb_time.tc  ActiveDisplayYMinimum=-49.42236160670042  ActiveDisplayYMaximum=444.75917558996025  DataLoggingVariableName=ScopeData15
  igbt power losses AFE Q2 : Scope  Commented=on  NumInputPorts=4
      settings: SampleTime=glb_time.tc  ActiveDisplayYMinimum=-81.375120798865652  ActiveDisplayYMaximum=732.47476633188421  DataLoggingVariableName=ScopeData26
  igbt power losses INV Q1 : Scope  Commented=on  NumInputPorts=4
      settings: SampleTime=glb_time.tc  ActiveDisplayYMinimum=427.7171442031123  ActiveDisplayYMaximum=1026.5989043156007  DataLoggingVariableName=ScopeData16
  igbt power losses INV Q2 : Scope  Commented=on  NumInputPorts=4
      settings: SampleTime=glb_time.tc  ActiveDisplayYMinimum=-115137.16014702634  ActiveDisplayYMaximum=1.0362344192177997E+6  DataLoggingVariableName=ScopeData27
  wires:
  From/1 -> igbt power losses AFE Q1/1  "igbt_ploss_afeQ1"
  From8/1 -> Bus Creator2/1  "igbt_JH_temp_invQ1"
  From60/1 -> Bus Creator10/1  "diode_JH_temp_invQ1"
  From45/1 -> Bus Creator7/2  "igbt_HA_temp_invQ2"
  From38/1 -> igbt power losses AFE Q2/2  "igbt_current_afeQ2"
  From36/1 -> igbt power losses AFE Q2/1  "igbt_ploss_afeQ2"
  From7/1 -> igbt power losses INV Q1/2  "igbt_current_invQ1"
  From3/1 -> Bus Creator1/1  "igbt_JH_temp_afeQ1"
  From43/1 -> igbt power losses INV Q2/2  "igbt_current_invQ2"
  From63/1 -> Bus Creator11/1  "diode_JH_temp_afeQ1"
  From9/1 -> Bus Creator2/2  "igbt_HA_temp_invQ1"
  From39/1 -> Bus Creator6/1  "igbt_JH_temp_afeQ2"
  Bus Creator11/1 -> diode power losses AFE Q1/2
  From59/1 -> diode power losses INV Q1/1  "diode_ploss_invQ1"
  From5/1 -> igbt power losses INV Q1/1  "igbt_ploss_invQ1"
  From40/1 -> Bus Creator6/2  "igbt_HA_temp_afeQ2"
  Bus Creator7/1 -> igbt power losses INV Q2/4
  From42/1 -> igbt power losses INV Q2/3  "igbt_voltage_invQ2"
  Bus Creator10/1 -> diode power losses INV Q1/2
  From44/1 -> Bus Creator7/1  "igbt_JH_temp_invQ2"
  From64/1 -> Bus Creator11/2  "diode_HA_temp_afeQ1"
  Bus Creator1/1 -> igbt power losses AFE Q1/4
  Bus Creator6/1 -> igbt power losses AFE Q2/4
  From1/1 -> igbt power losses AFE Q1/3  "igbt_voltage_afeQ1"
  From2/1 -> igbt power losses AFE Q1/2  "igbt_current_afeQ1"
  From4/1 -> Bus Creator1/2  "igbt_HA_temp_afeQ1"
  From62/1 -> diode power losses AFE Q1/1  "diode_ploss_afeQ1"
  Bus Creator2/1 -> igbt power losses INV Q1/4
  From61/1 -> Bus Creator10/2  "diode_HA_temp_invQ1"
  From6/1 -> igbt power losses INV Q1/3  "igbt_voltage_invQ1"
  From41/1 -> igbt power losses INV Q2/1  "igbt_ploss_invQ2"
  From37/1 -> igbt power losses AFE Q2/3  "igbt_voltage_afeQ2"

== system afe_inv_psm_with_hf_models/scopes/machine_side ==
  Bus Creator3 : BusCreator  Inputs=2
  Bus Creator4 : BusCreator  Inputs=2
  Bus Creator5 : BusCreator  Inputs=2
  From56 : From  Commented=on  GotoTag=inverter_voltage_ee_phase_u
  From57 : From  Commented=on  GotoTag=inverter_voltage_ee_phase_v
  From58 : From  Commented=on  GotoTag=inverter_voltage_ee_phase_w
  Gain1 : Gain  Gain=1e-3
  LTI System : cstblocks_lti/LTI System  sys=filters.inv.SOF_50Hz.ss_c  IC=[]  PadeOrder=0
  LTI System1 : cstblocks_lti/LTI System  sys=filters.inv.SOF_50Hz.ss_c  IC=[]  PadeOrder=0
  inverter_voltage_ee : Scope  Commented=on  NumInputPorts=3
      settings: SampleTime=tc  ActiveDisplayYMinimum=-207.5782073641667  ActiveDisplayYMaximum=1301.7632755987056  DataLoggingVariableName=ScopeData30
  is_uvw/us_uvw : Scope  NumInputPorts=2
      settings: SampleTime=glb_time.tc  ActiveDisplayYMinimum=-1.2325569675038333  ActiveDisplayYMaximum=1.2339333833020862  DataLoggingVariableName=ScopeData25
  motor currents : Scope  NumInputPorts=3
      settings: SampleTime=glb_time.tc  ActiveDisplayYMinimum=-232.58671124644178  ActiveDisplayYMaximum=232.76282128626991  DataLoggingVariableName=ScopeData17
  motor dq : Scope  NumInputPorts=2
      settings: SampleTime=glb_time.tc  ActiveDisplayYMinimum=-850.02239826316088  ActiveDisplayYMaximum=207.16586596148719  DataLoggingVariableName=ScopeData18
  motor mech : Scope  NumInputPorts=3
      settings: SampleTime=glb_time.tc  ActiveDisplayYMinimum=-2.216582738378952  ActiveDisplayYMaximum=19.949244645410573  DataLoggingVariableName=ScopeData11
  phi_alpha_pmsm/phi_beta_pmsm : Scope  NumInputPorts=2
      settings: SampleTime=glb_time.tc  ActiveDisplayYMinimum=-4.8008048511588592  ActiveDisplayYMaximum=4.8008564448893649  DataLoggingVariableName=ScopeData19
  wires:
  [iu_psm] -> motor currents/1  "iu_psm"
  [psi_r_beta_psm] -> phi_alpha_pmsm/phi_beta_pmsm/2
  [id_psm] -> Bus Creator4/2  "id_psm"
  [ud_psm] -> Bus Creator3/1  "ud_psm"
  Bus Creator4/1 -> motor dq/2
  [iq_psm] -> Bus Creator4/1  "iq_psm"
  [uq_psm] -> Bus Creator3/2  "uq_psm"
  Bus Creator3/1 -> motor dq/1
  [psi_r_alpha_psm] -> phi_alpha_pmsm/phi_beta_pmsm/1
  [iv_psm] -> motor currents/2  "iv_psm"
  [iw_psm] -> motor currents/3  "iw_psm"
  [pwr_in_psm] -> LTI System/1
  LTI System1/1 -> Bus Creator5/2  "pwr_out_psm (kW)"
  [torque_load_psm] -> Gain1/1
  LTI System/1 -> Bus Creator5/1  "pin_psm (kW)"
  Gain1/1 -> motor mech/2  "torque_load_psm (kNm)"
  [rpm_motor] -> motor mech/1  "omega_elec_psm (rpm)"
  Bus Creator5/1 -> motor mech/3
  [pwr_out_psm] -> LTI System1/1
  [us_uvw_pu] -> is_uvw/us_uvw/2  "us_uvw_pu_mod1"
  [is_uvw_pu] -> is_uvw/us_uvw/1  "is_uvw_pu_mod1"
  From58/1 -> inverter_voltage_ee/3  "inverter_voltage_ee_phase_w"
  From56/1 -> inverter_voltage_ee/1  "inverter_voltage_ee_phase_u"
  From57/1 -> inverter_voltage_ee/2  "inverter_voltage_ee_phase_v"

== system afe_inv_psm_with_hf_models/scopes/mosfet_power_losses ==
  Bus Creator8 : BusCreator  Commented=on  Inputs=2
  Bus Creator9 : BusCreator  Commented=on  Inputs=2
  From46 : From  Commented=on  GotoTag=mosfet_ploss_invQ1
  From47 : From  Commented=on  GotoTag=mosfet_voltage_invQ1
  From48 : From  Commented=on  GotoTag=mosfet_current_invQ1
  From49 : From  Commented=on  GotoTag=mosfet_JH_temp_invQ1
  From50 : From  Commented=on  GotoTag=mosfet_HA_temp_invQ1
  From51 : From  Commented=on  GotoTag=mosfet_ploss_invQ2
  From52 : From  Commented=on  GotoTag=mosfet_voltage_invQ2
  From53 : From  Commented=on  GotoTag=mosfet_current_invQ2
  From54 : From  Commented=on  GotoTag=mosfet_JH_temp_invQ2
  From55 : From  Commented=on  GotoTag=mosfet_HA_temp_invQ2
  mosfet power losses INV Q1 : Scope  Commented=on  NumInputPorts=4
      settings: SampleTime=glb_time.tc  ActiveDisplayYMinimum=-52.647210306071649  ActiveDisplayYMaximum=473.81757031333393  DataLoggingVariableName=ScopeData28
  mosfet power losses INV Q2 : Scope  Commented=on  NumInputPorts=4
      settings: SampleTime=glb_time.tc  ActiveDisplayYMinimum=-60.051099059926763  ActiveDisplayYMaximum=540.45256909803  DataLoggingVariableName=ScopeData29
  wires:
  From53/1 -> mosfet power losses INV Q2/3  "mosfet_current_invQ2"
  From47/1 -> mosfet power losses INV Q1/2  "mosfet_voltage_invQ1"
  From55/1 -> Bus Creator9/2  "mosfet_HA_temp_invQ2"
  From54/1 -> Bus Creator9/1  "mosfet_JH_temp_invQ2"
  From46/1 -> mosfet power losses INV Q1/1  "mosfet_ploss_invQ1"
  From50/1 -> Bus Creator8/2  "mosfet_HA_temp_invQ1"
  From48/1 -> mosfet power losses INV Q1/3  "mosfet_current_invQ1"
  Bus Creator8/1 -> mosfet power losses INV Q1/4
  From52/1 -> mosfet power losses INV Q2/2  "mosfet_voltage_invQ2"
  From51/1 -> mosfet power losses INV Q2/1  "mosfet_ploss_invQ2"
  Bus Creator9/1 -> mosfet power losses INV Q2/4
  From49/1 -> Bus Creator8/1  "mosfet_JH_temp_invQ1"
